simulink subsystem "pwm_to_force"  (R2026a)
settings: Solver=VariableStepAuto
undefined symbols (not defined in the file): P, S
PreSaveFcn:
  | defaultToFileBlockNames(bdroot);
settings Model: DefaultTestHarness=pwm_to_force_Harness1  Creator=koryh  LastModifiedBy=kjhaydon

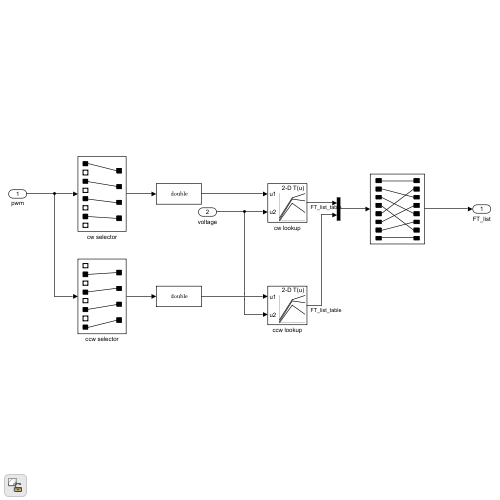
[thumbnail: Simulink's stored preview of the top-level diagram]
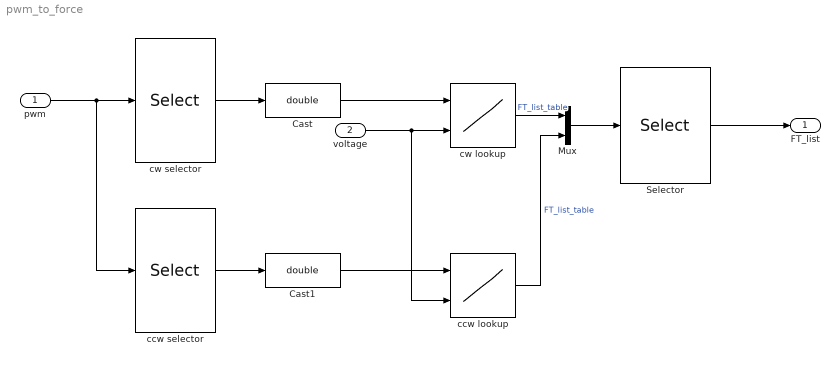
== system pwm_to_force ==
  pwm : Inport  SampleTime=S.dt_control
  voltage : Inport  Port=2
  Cast : DataTypeConversion  OutDataTypeStr=double  SaturateOnIntegerOverflow=off  RndMeth=Floor
  Cast1 : DataTypeConversion  OutDataTypeStr=double  SaturateOnIntegerOverflow=off  RndMeth=Floor
  Mux : Mux  Inputs=2
  Selector : Selector  InputPortWidth=8  IndexOptions=Index vector (dialog)  Indices=[1 5 2 6 3 7 4 8]  OutputSizes=1
  ccw lookup : Lookup_n-D  BreakpointsForDimension1=flip(P.Constants.ccw_pwm)  BreakpointsForDimension2=P.Constants.voltage  Table=flip(P.Constants.ccw_force,1)  ExtrapMethod=Clip  UseLastTableValue=on  InternalRulePriority=Speed  RndMeth=Simplest
      settings: InputPortMap=u0,u1
  ccw selector : Selector  InputPortWidth=8  IndexOptions=Index vector (dialog)  Indices=[2 4 6 8]  OutputSizes=1
  cw lookup : Lookup_n-D  BreakpointsForDimension1=P.Constants.cw_pwm  BreakpointsForDimension2=P.Constants.voltage  Table=P.Constants.cw_force  ExtrapMethod=Clip  UseLastTableValue=on  InternalRulePriority=Speed  RndMeth=Simplest
      settings: InputPortMap=u0,u1
  cw selector : Selector  InputPortWidth=8  IndexOptions=Index vector (dialog)  Indices=[1 3 5 7]  OutputSizes=1
  FT_list : Outport
  wires:
  voltage/1 -> cw lookup/2, ccw lookup/2
  Cast/1 -> cw lookup/1
  pwm/1 -> ccw selector/1, cw selector/1
  cw selector/1 -> Cast/1
  ccw selector/1 -> Cast1/1
  Cast1/1 -> ccw lookup/1
  cw lookup/1 -> Mux/1  "FT_list_table"
  Mux/1 -> Selector/1
  ccw lookup/1 -> Mux/2  "FT_list_table"
  Selector/1 -> FT_list/1
